simulink model "heatdrive_ecc_coupled_se21"  (R2025b)
settings: Solver=ode23t  StartTime=0.0  StopTime=10  FixedStep=0.1  MaxStep=0.4  RelTol=1e-2  AbsTol=1e-3
values from neighbouring files (symbols this model uses):
  cold_load_heat_W = 0.0    (= 0)    [Build_Simulink_Exchange_Params.m]
  cold_load_T_init = get_stage_field(stage_config, 'cold_load_T_in', get_stage_field(stage_config,          'chip_T_in', get_option_field(exchange_options, 'cold_load_T_init', get_option_field(exchange_options, 'chip_T_init', 293.0))))    [Build_Simulink_Exchange_Params.m]    (also in Create_Simulink_Exchange_Runtime.m = get_option_field(options, 'cold_load_T_init',          get_o)
  cold_sink_T_init = get_stage_field(stage_config, 'cold_sink_T_in', get_option_field(exchange_options, 'cold_sink_T_init', 293.0))    [Build_Simulink_Exchange_Params.m]    (also in Create_Simulink_Exchange_Runtime.m = get_option_field(options, 'cold_sink_T_init', ambient_T_init)
  hot_sink_T_init = get_stage_field(stage_config, 'hot_sink_T_in', get_option_field(exchange_options, 'hot_sink_T_init', 293.0))    [Build_Simulink_Exchange_Params.m]    (also in Create_Simulink_Exchange_Runtime.m = get_option_field(options, 'hot_sink_T_init', ambient_T_init))
  mdot_cooldown_source_kgps = mdot_target_kgps    [Build_Simulink_Exchange_Params.m]
  mdot_hold_source_kgps = mdot_target_kgps    [Build_Simulink_Exchange_Params.m]
  pressure_pi_bias_MPa = pressure_pi_dp_guess_MPa    [Build_Simulink_Exchange_Params.m]
  pressure_pi_error_filter_tau_s = max(get_option_field(exchange_options, 'pressure_pi_error_filter_tau_s', 0.002), 1.0e-5)    [Build_Simulink_Exchange_Params.m]
  pressure_pi_error_normalization_gain_kgps_inv = 1.0    (= 1)    [Build_Simulink_Exchange_Params.m]
  pressure_pi_max_MPa = pressure_pi_dp_guess_MPa + pressure_pi_margin_MPa    [Build_Simulink_Exchange_Params.m]
  shex_sink_T_init = get_option_field(exchange_options, 'shex_sink_T_init', hot_sink_T_init)    [Build_Simulink_Exchange_Params.m]
undefined symbols (not defined in the file or in its folder): constitutive_sample_time_s, constitutive_state21_initial, se_constitutive_T21_initial, se_pressure_integrator_max_MPa, se_pressure_pi_ki_MPa_per_kgps_s, se_pressure_pi_kp_MPa_per_kgps, se_pressure_pi_min_MPa, se_solver_T_init_21_internal, se_stage2_pressure_integrator_min_MPa, se_stage4_pressure_integrator_min_MPa, sma_constitutive_T21_initial, sma_mdot_stage1_source_kgps, sma_mdot_stage3_source_kgps, sma_pressure_integrator_max_MPa, sma_pressure_integrator_min_MPa, sma_pressure_pi_ki_MPa_per_kgps_s, sma_pressure_pi_kp_MPa_per_kgps, sma_pressure_pi_min_MPa, sma_solver_T_init_21_internal
libraries: fl_lib x484, nesl_utility x232, SimscapeFluids_lib x20
(part 3 of 8)

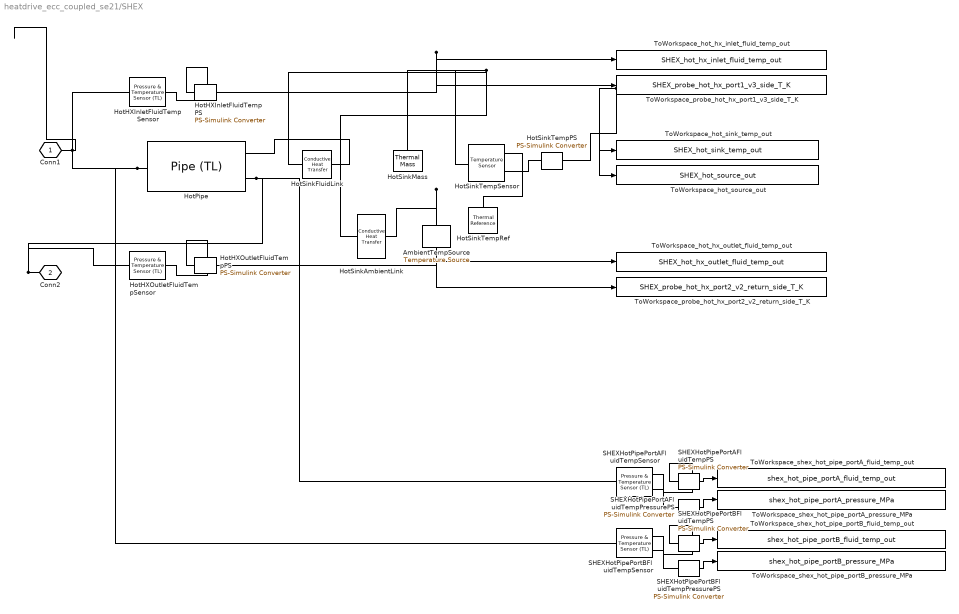
== system heatdrive_ecc_coupled_se21/SHEX ==
  AmbientTempSource : fl_lib/Thermal/Thermal Sources/Temperature Source  temperature=shex_source_T_init K
  HotHXInletFluidTempPS : nesl_utility/PS-Simulink Converter  PhysicalDomain=network_engine_domain  SubClassName=ps_output  LeftPortType=input  RightPortType=output  PseudoPeriodic=off  Frequencies=[]  VectorFormat=1-D array  Unit=K  AffineConversion=off
  HotHXInletFluidTempSensor : fl_lib/Thermal Liquid/Sensors/Pressure & Temperature Sensor (TL)  reference=foundation.enum.MeasurementReference.absolute  pressure=false  pressure_spec=foundation.enum.PressureMeasementSpec.Absolute  temperature=true
      settings: InternalSimscapePortConfiguration="{\"Bottom\":[{\"id\":\"T\",\"label\":\"T\",\"type\":\"output\"}],\"Left\":[{\"id\":\"A\",\"label\":\"A\",\"type\":\"foundation.thermal_liquid.thermal_liquid\"}],\"Right\":[],\"Top\":[]}"
  HotHXOutletFluidTempPS : nesl_utility/PS-Simulink Converter  PhysicalDomain=network_engine_domain  SubClassName=ps_output  LeftPortType=input  RightPortType=output  PseudoPeriodic=off  Frequencies=[]  VectorFormat=1-D array  Unit=K  AffineConversion=off
  HotHXOutletFluidTempSensor : fl_lib/Thermal Liquid/Sensors/Pressure & Temperature Sensor (TL)  reference=foundation.enum.MeasurementReference.absolute  pressure=false  pressure_spec=foundation.enum.PressureMeasementSpec.Absolute  temperature=true
      settings: InternalSimscapePortConfiguration="{\"Bottom\":[{\"id\":\"T\",\"label\":\"T\",\"type\":\"output\"}],\"Left\":[{\"id\":\"A\",\"label\":\"A\",\"type\":\"foundation.thermal_liquid.thermal_liquid\"}],\"Right\":[],\"Top\":[]}"
  HotPipe : fl_lib/Thermal Liquid/Elements/Pipe (TL)  length=tube_l m  area=sma_pipe_fa m^2  Dh=D_e m  length_add=0 m  roughness=15e-6 m  Re_lam=2000  Re_tur=4000  shape_factor=64  Nu_lam=nuh  dynamic_compressibility=false  inertia=false  p0=1 MPa  T0=shex_hot_side_fluid_T_init K  mdot0=0 kg/s  p_nominal=1 MPa  T_nominal=293.15 K
  HotSinkAmbientLink : fl_lib/Thermal/Thermal Elements/Conductive Heat Transfer  thermal_type=foundation.enum.ConstantVariableTabulated.Constant  wall_geometry=foundation.enum.ConductionWallGeometry.Planar  area=1 m^2  thickness=1 m  d_in=0.05 m  d_out=0.1 m  L=1 m  th_cond_min=10 W/(K*m)  th_cond=shex_sink_ambient_G_W_per_K W/(K*m)  th_cond_TLU=[413, 401, 392, 383, 371, 357, 342] W/(K*m)  temp_TLU=[200, 273, 400, 600, 800, 1000, 1200] K  T_specify=off  T_priority=None  T=0 K  T_nominal_specify=off  T_nominal_value=1  T_nominal_unit=K  Q_specify=off  Q_priority=None  Q=0 W  Q_nominal_specify=off  Q_nominal_value=1  Q_nominal_unit=W
  HotSinkFluidLink : fl_lib/Thermal/Thermal Elements/Conductive Heat Transfer  thermal_type=foundation.enum.ConstantVariableTabulated.Constant  wall_geometry=foundation.enum.ConductionWallGeometry.Planar  area=1 m^2  thickness=1 m  d_in=0.05 m  d_out=0.1 m  L=1 m  th_cond_min=10 W/(K*m)  th_cond=shex_sink_fluid_G_W_per_K W/(K*m)  th_cond_TLU=[413, 401, 392, 383, 371, 357, 342] W/(K*m)  temp_TLU=[200, 273, 400, 600, 800, 1000, 1200] K  T_specify=off  T_priority=None  T=0 K  T_nominal_specify=off  T_nominal_value=1  T_nominal_unit=K  Q_specify=off  Q_priority=None  Q=0 W  Q_nominal_specify=off  Q_nominal_value=1  Q_nominal_unit=W
  HotSinkMass : fl_lib/Thermal/Thermal Elements/Thermal Mass  mass_type=foundation.enum.constant_variable.constant  mass=shex_sink_mass_kg kg  sp_heat=thermal_mass_cp_ref J/(K*kg)  mass_min=1e-6 kg  num_ports=foundation.enum.numPorts2.one  m_specify=off  m_priority=High  m=1 kg  m_nominal_specify=off  m_nominal_value=1  m_nominal_unit=kg  T_specify=on  T_priority=High  T=shex_sink_T_init K  T_nominal_specify=off  T_nominal_value=1  T_nominal_unit=K  Q_specify=off  Q_priority=None  Q=0 W  Q_nominal_specify=off  Q_nominal_value=1  Q_nominal_unit=W
  HotSinkTempPS : nesl_utility/PS-Simulink Converter  PhysicalDomain=network_engine_domain  SubClassName=ps_output  LeftPortType=input  RightPortType=output  PseudoPeriodic=off  Frequencies=[]  VectorFormat=1-D array  Unit=K  AffineConversion=off
  HotSinkTempRef : fl_lib/Thermal/Thermal Elements/Thermal Reference
  HotSinkTempSensor : fl_lib/Thermal/Thermal Sensors/Temperature Sensor  temperature_measure=foundation.enum.MeasurementReference.difference
  SHEXHotPipePortAFluidTempPS : nesl_utility/PS-Simulink Converter  PhysicalDomain=network_engine_domain  SubClassName=ps_output  LeftPortType=input  RightPortType=output  PseudoPeriodic=off  Frequencies=[]  VectorFormat=1-D array  Unit=K  AffineConversion=off
  SHEXHotPipePortAFluidTempPressurePS : nesl_utility/PS-Simulink Converter  PhysicalDomain=network_engine_domain  SubClassName=ps_output  LeftPortType=input  RightPortType=output  PseudoPeriodic=off  Frequencies=[]  VectorFormat=1-D array  Unit=MPa  AffineConversion=off
  SHEXHotPipePortAFluidTempSensor : fl_lib/Thermal Liquid/Sensors/Pressure & Temperature Sensor (TL)  reference=foundation.enum.MeasurementReference.absolute  pressure=true  pressure_spec=foundation.enum.PressureMeasementSpec.Absolute  temperature=true
      settings: InternalSimscapePortConfiguration="{\"Bottom\":[{\"id\":\"T\",\"label\":\"T\",\"type\":\"output\"}],\"Left\":[{\"id\":\"A\",\"label\":\"A\",\"type\":\"foundation.thermal_liquid.thermal_liquid\"}],\"Right\":[{\"id\":\"Pa\",\"label\":\"Pa\",\"type\":\"output\"}],\"Top\":[]}"
  SHEXHotPipePortBFluidTempPS : nesl_utility/PS-Simulink Converter  PhysicalDomain=network_engine_domain  SubClassName=ps_output  LeftPortType=input  RightPortType=output  PseudoPeriodic=off  Frequencies=[]  VectorFormat=1-D array  Unit=K  AffineConversion=off
  SHEXHotPipePortBFluidTempPressurePS : nesl_utility/PS-Simulink Converter  PhysicalDomain=network_engine_domain  SubClassName=ps_output  LeftPortType=input  RightPortType=output  PseudoPeriodic=off  Frequencies=[]  VectorFormat=1-D array  Unit=MPa  AffineConversion=off
  SHEXHotPipePortBFluidTempSensor : fl_lib/Thermal Liquid/Sensors/Pressure & Temperature Sensor (TL)  reference=foundation.enum.MeasurementReference.absolute  pressure=true  pressure_spec=foundation.enum.PressureMeasementSpec.Absolute  temperature=true
      settings: InternalSimscapePortConfiguration="{\"Bottom\":[{\"id\":\"T\",\"label\":\"T\",\"type\":\"output\"}],\"Left\":[{\"id\":\"A\",\"label\":\"A\",\"type\":\"foundation.thermal_liquid.thermal_liquid\"}],\"Right\":[{\"id\":\"Pa\",\"label\":\"Pa\",\"type\":\"output\"}],\"Top\":[]}"
  ToWorkspace_hot_hx_inlet_fluid_temp_out : ToWorkspace  VariableName=SHEX_hot_hx_inlet_fluid_temp_out  SaveFormat=Structure With Time  SampleTime=-1
  ToWorkspace_hot_hx_outlet_fluid_temp_out : ToWorkspace  VariableName=SHEX_hot_hx_outlet_fluid_temp_out  SaveFormat=Structure With Time  SampleTime=-1
  ToWorkspace_hot_sink_temp_out : ToWorkspace  VariableName=SHEX_hot_sink_temp_out  SaveFormat=Structure With Time  SampleTime=-1
  ToWorkspace_hot_source_out : ToWorkspace  VariableName=SHEX_hot_source_out  SaveFormat=Structure With Time  SampleTime=-1
  ToWorkspace_probe_hot_hx_port1_v3_side_T_K : ToWorkspace  VariableName=SHEX_probe_hot_hx_port1_v3_side_T_K  SaveFormat=Structure With Time  SampleTime=-1
  ToWorkspace_probe_hot_hx_port2_v2_return_side_T_K : ToWorkspace  VariableName=SHEX_probe_hot_hx_port2_v2_return_side_T_K  SaveFormat=Structure With Time  SampleTime=-1
  ToWorkspace_shex_hot_pipe_portA_fluid_temp_out : ToWorkspace  VariableName=shex_hot_pipe_portA_fluid_temp_out  SaveFormat=Structure With Time  SampleTime=-1
  ToWorkspace_shex_hot_pipe_portA_pressure_MPa : ToWorkspace  VariableName=shex_hot_pipe_portA_pressure_MPa  SaveFormat=Structure With Time  SampleTime=-1
  ToWorkspace_shex_hot_pipe_portB_fluid_temp_out : ToWorkspace  VariableName=shex_hot_pipe_portB_fluid_temp_out  SaveFormat=Structure With Time  SampleTime=-1
  ToWorkspace_shex_hot_pipe_portB_pressure_MPa : ToWorkspace  VariableName=shex_hot_pipe_portB_pressure_MPa  SaveFormat=Structure With Time  SampleTime=-1
  Conn1 : PMIOPort  Side=Right
  Conn2 : PMIOPort  Port=2  Side=Left
  wires:
  HotHXOutletFluidTempPS/1 -> ToWorkspace_probe_hot_hx_port2_v2_return_side_T_K/1, ToWorkspace_hot_hx_outlet_fluid_temp_out/1
  HotHXInletFluidTempPS/1 -> ToWorkspace_probe_hot_hx_port1_v3_side_T_K/1, ToWorkspace_hot_hx_inlet_fluid_temp_out/1
  HotSinkTempPS/1 -> ToWorkspace_hot_source_out/1, ToWorkspace_hot_sink_temp_out/1
  SHEXHotPipePortAFluidTempPS/1 -> ToWorkspace_shex_hot_pipe_portA_fluid_temp_out/1
  SHEXHotPipePortAFluidTempPressurePS/1 -> ToWorkspace_shex_hot_pipe_portA_pressure_MPa/1
  SHEXHotPipePortBFluidTempPS/1 -> ToWorkspace_shex_hot_pipe_portB_fluid_temp_out/1
  SHEXHotPipePortBFluidTempPressurePS/1 -> ToWorkspace_shex_hot_pipe_portB_pressure_MPa/1
  connections:
  HotHXOutletFluidTempSensor/RConn1 -- HotHXOutletFluidTempPS/LConn1
  HotHXInletFluidTempSensor/RConn1 -- HotHXInletFluidTempPS/LConn1
  HotSinkAmbientLink/RConn1 -- AmbientTempSource/LConn1
  HotSinkTempSensor/RConn2 -- HotSinkTempPS/LConn1
  HotSinkTempSensor/RConn1 -- HotSinkTempRef/LConn1
  HotSinkFluidLink/RConn1 -- HotPipe/LConn2
  HotSinkAmbientLink/LConn1 -- HotSinkTempSensor/LConn1 -- HotSinkMass/LConn1 -- HotSinkFluidLink/LConn1
  HotHXOutletFluidTempSensor/LConn1 -- HotPipe/LConn1 -- SHEXHotPipePortAFluidTempSensor/LConn1 -- Conn2/RConn1
  HotHXInletFluidTempSensor/LConn1 -- HotPipe/RConn1 -- SHEXHotPipePortBFluidTempSensor/LConn1 -- Conn1/RConn1
  SHEXHotPipePortAFluidTempSensor/RConn2 -- SHEXHotPipePortAFluidTempPS/LConn1
  SHEXHotPipePortAFluidTempSensor/RConn1 -- SHEXHotPipePortAFluidTempPressurePS/LConn1
  SHEXHotPipePortBFluidTempSensor/RConn2 -- SHEXHotPipePortBFluidTempPS/LConn1
  SHEXHotPipePortBFluidTempSensor/RConn1 -- SHEXHotPipePortBFluidTempPressurePS/LConn1
